simulink model "flow_4d"  (R2025a)
settings: Solver=VariableStepAuto  StartTime=0.0  StopTime=10.0  RelTol=1e-3
values from neighbouring files (symbols this model uses):
  B = 21.8    [calc_task2.m]    (also in pseudocde_4d.m = 0; ship.m)
  C_RB = 0    [pseudocde_4d.m]
  delta_c = 0.1    [main.m]    (also in ship.m = sign(delta_c)*delta_max)
  M_RB_inv = 0    [pseudocde_4d.m]
  n_c = (30/pi) * simdata(:,10)    [main.m]    (also in ship.m = u(2))
settings Model: Creator=mathi  LastModifiedBy=mathi

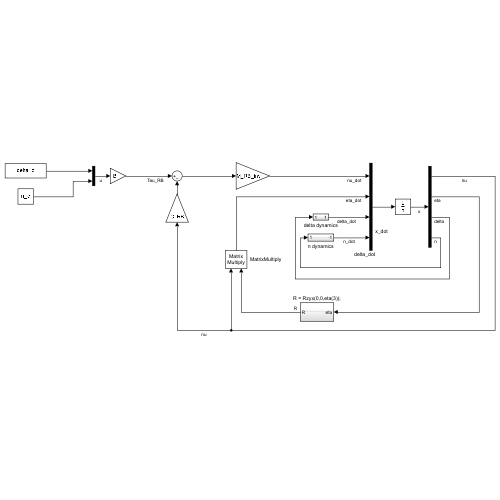
[thumbnail: Simulink's stored preview of the top-level diagram]
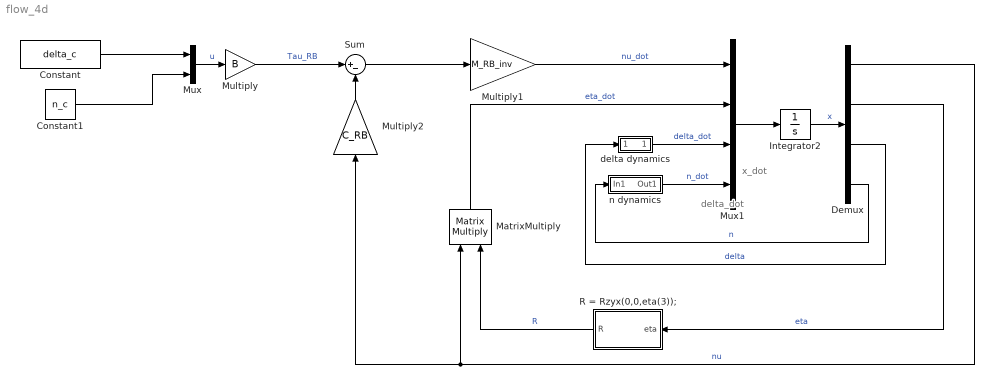
== system flow_4d ==
  note: delta_dot
  note: x_dot
  Constant : Constant  Value=delta_c
  Constant1 : Constant  Value=n_c
  Demux : Demux
  Integrator2 : Integrator
  MatrixMultiply : Product  Multiplication=Matrix(*)
  Multiply : Gain  Gain=B
  Multiply1 : Gain  Gain=M_RB_inv
  Multiply2 : Gain  Gain=C_RB
  Mux : Mux  Inputs=2
  Mux1 : Mux
  R = Rzyx(0,0,eta(3)); : Subsystem
  Sum : Sum  Inputs=|+-
  delta dynamics : Subsystem
  n dynamics : Subsystem
  wires:
  Constant1/1 -> Mux/2
  Constant/1 -> Mux/1
  Mux/1 -> Multiply/1  "u"
  Multiply/1 -> Sum/1  "Tau_RB"
  Multiply2/1 -> Sum/2
  Sum/1 -> Multiply1/1
  Multiply1/1 -> Mux1/1  "nu_dot"
  Demux/1 -> Multiply2/1, MatrixMultiply/1  "nu"
  R = Rzyx(0,0,eta(3));/1(R) -> MatrixMultiply/2  "R"
  Mux1/1 -> Integrator2/1
  Integrator2/1 -> Demux/1  "x"
  Demux/2 -> R = Rzyx(0,0,eta(3));/1(eta)  "eta"
  delta dynamics/1(Out1) -> Mux1/3  "delta_dot"
  n dynamics/1(Out1) -> Mux1/4  "n_dot"
  Demux/3 -> delta dynamics/1(In1)  "delta"
  Demux/4 -> n dynamics/1(In1)  "n"
  MatrixMultiply/1 -> Mux1/2  "eta_dot"

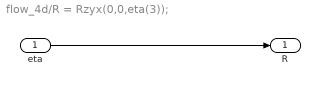
== system flow_4d/R = Rzyx(0,0,eta(3)); ==
  eta : Inport
  R : Outport
  wires:
  eta/1 -> R/1

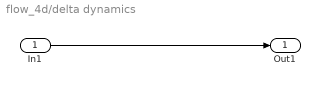
== system flow_4d/delta dynamics ==
  In1 : Inport
  Out1 : Outport
  wires:
  In1/1 -> Out1/1

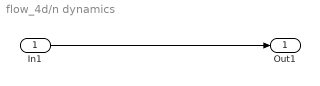
== system flow_4d/n dynamics ==
  In1 : Inport
  Out1 : Outport
  wires:
  In1/1 -> Out1/1
